simulink model "Sim2Real_ankle_motion_2025a"  (R2025a)
settings: Solver=FixedStepDiscrete  StartTime=0.0  StopTime=8  FixedStep=Ts_1ms  MaxStep=0.002  RelTol=1e-3
InitFcn:
  | modelFile = get_param(bdroot,'FileName');
  | if isempty(modelFile)
  |     error('The model must be saved before running InitFcn.');
  | end
  | 
  | % Folder where the .slx model is located
  | modelFolder = fileparts(char(modelFile));
  | 
  | % Find the parent folder named "resources" by going upwards
  | currentFolder  = modelFolder;
  | materialFolder = '';
  | 
  | while true
  |     [parentFolder, currentName] = fileparts(currentFolder);
  | 
  |     if strcmpi(currentName, 'resources')
  |         materialFolder = currentFolder;
  |         break;
  |     end
  | 
  |     if strcmp(parentFolder, currentFolder)
  |         error('Could not find a parent folder named "resources" starting from: %s', modelFolder);
  |     end
  | 
  |     currentFolder = parentFolder;
  | end
  | 
  | % Search recursively for the MuJoCo XML inside "material"
  | xmlSearch = dir(fullfile(materialFolder, '**', 'unitree_G1.xml'));
  | 
  | if isempty(xmlSearch)
  |     error('MuJoCo XML file not found inside material folder: %s', materialFolder);
  | elseif numel(xmlSearch) > 1
  |     error('Multiple unitree_G1.xml files found inside material folder. Leave only one valid XML.');
  | end
  | 
  | mujocoFolder = xmlSearch(1).folder;
  | xmlFullPath  = fullfile(xmlSearch(1).folder, xmlSearch(1).name);
  | 
  | % Save in base workspace in case you want to inspect them
  | assignin('base','modelFolder',modelFolder);
  | assignin('base','materialFolder',materialFolder);
  | assignin('base','mujocoFolder',mujocoFolder);
  | assignin('base','xmlFullPath',xmlFullPath);
  | 
  | % Final existence check
  | if exist(xmlFullPath,'file') ~= 2
  |     error('MuJoCo XML file not found: %s', xmlFullPath);
  | end
  | 
  | % Add the XML folder to the path so WHICH can find it
  | addpath(mujocoFolder, '-begin');
  | rehash path;
  | 
  | % Run launcher from the same folder as the model
  | launcherFile = fullfile(modelFolder, 'launcher_ankle_motion.mlx');
  | if exist(launcherFile,'file') == 2
  |     run(launcherFile);
  | else
  |     error('Launcher file not found: %s', launcherFile);
  | ... (+17 lines)
StopFcn:
  | drawnow; pause(0.05);
  | 
  | % Stop figures
  | tags = {'G1_IMUState','G1_MotorState'};
  | for k = 1:numel(tags)
  |     delete(findall(0,'Type','uifigure','Tag',tags{k}));
  |     delete(findall(0,'Type','figure' , 'Tag',tags{k}));
  | end
  | 
  | 
  | % Automatic ankle metrics CSV (installed once)
  | addpath(fileparts(get_param('Sim2Real_ankle_motion_2025a', 'FileName')));
  | ankle_motion_csv('save');
undefined symbols (not defined in the file or in its folder): crc, DiscIntNeverNeededParam, mode_machine, mode_pr, motor_cmd, reserve, Ts_1ms
libraries: ros2lib x3, slpidlib x1, mjLib x1
(part 2 of 2)

== matlab function Sim2Real_ankle_motion_2025a/SIM2REAL VARIANT SUBSYSTEM/ROS 2 SUBSYSTEM/ROS 2 SUBSYSTEM/JOINT COMMAND/BUILD motor_cmd BUS ==
  data: motor_cmd output Bus: SL_Bus_unitree_hg_MotorCmd; bus_tau_ref input Bus: bus_tau_ref; bus_pos_ref input Bus: bus_pos_ref; bus_vel_ref input Bus: bus_vel_ref; bus_kp_kd_dyn input Bus: bus_kp_kd_dyn
function motor_cmd = g1_build_motorcmd_vectors( ...
    bus_tau_ref, bus_pos_ref, bus_vel_ref, bus_kp_kd_dyn)
%#codegen

N     = int32(35);   
NBODY = int32(29);   
NLL = int32(6);   % left leg
NRL = int32(6);   % right leg
NW  = int32(3);   % waist
NLA = int32(7);   % left arm
NRA = int32(7);   % right arm

% tau refs
left_leg_tau_ref   = bus_tau_ref.left_leg_tau_ref;
right_leg_tau_ref  = bus_tau_ref.right_leg_tau_ref;
waist_tau_ref      = bus_tau_ref.waist_tau_ref;
left_arm_tau_ref   = bus_tau_ref.left_arm_tau_ref;
right_arm_tau_ref  = bus_tau_ref.right_arm_tau_ref;

% pos refs
left_leg_pos_ref   = bus_pos_ref.left_leg_pos_ref;
right_leg_pos_ref  = bus_pos_ref.right_leg_pos_ref;
waist_pos_ref      = bus_pos_ref.waist_pos_ref;
left_arm_pos_ref   = bus_pos_ref.left_arm_pos_ref;
right_arm_pos_ref  = bus_pos_ref.right_arm_pos_ref;

% vel refs
left_leg_vel_ref   = bus_vel_ref.left_leg_vel_ref;
right_leg_vel_ref  = bus_vel_ref.right_leg_vel_ref;
waist_vel_ref      = bus_vel_ref.waist_vel_ref;
left_arm_vel_ref   = bus_vel_ref.left_arm_vel_ref;
right_arm_vel_ref  = bus_vel_ref.right_arm_vel_ref;

% gains
left_leg_kp_kd     = bus_kp_kd_dyn.left_leg_kp_kd_dyn;
right_leg_kp_kd    = bus_kp_kd_dyn.right_leg_kp_kd_dyn;
waist_kp_kd        = bus_kp_kd_dyn.waist_kp_kd_dyn;
left_arm_kp_kd     = bus_kp_kd_dyn.left_arm_kp_kd_dyn;
right_arm_kp_kd    = bus_kp_kd_dyn.right_arm_kp_kd_dyn;

% Force shapes (column) and types
ll_q   = single(left_leg_pos_ref(:));   rl_q   = single(right_leg_pos_ref(:));
w_q    = single(waist_pos_ref(:));
la_q   = single(left_arm_pos_ref(:));   ra_q   = single(right_arm_pos_ref(:));

ll_dq  = single(left_leg_vel_ref(:));   rl_dq  = single(right_leg_vel_ref(:));
w_dq   = single(waist_vel_ref(:));
la_dq  = single(left_arm_vel_ref(:));   ra_dq  = single(right_arm_vel_ref(:));

ll_tau = single(left_leg_tau_ref(:));   rl_tau = single(right_leg_tau_ref(:));
w_tau  = single(waist_tau_ref(:));
la_tau = single(left_arm_tau_ref(:));   ra_tau = single(right_arm_tau_ref(:));

% Validate input sizes 
ok_ll = (int32(numel(ll_q))  == NLL) && (int32(numel(ll_dq))  == NLL) && (int32(numel(ll_tau))  == NLL);
ok_rl = (int32(numel(rl_q))  == NRL) && (int32(numel(rl_dq))  == NRL) && (int32(numel(rl_tau))  == NRL);
ok_w  = (int32(numel(w_q))   == NW ) && (int32(numel(w_dq))   == NW ) && (int32(numel(w_tau))   == NW );
ok_la = (int32(numel(la_q))  == NLA) && (int32(numel(la_dq))  == NLA) && (int32(numel(la_tau))  == NLA);
ok_ra = (int32(numel(ra_q))  == NRA) && (int32(numel(ra_dq))  == NRA) && (int32(numel(ra_tau))  == NRA);

% Gains: (6x2,6x2,3x2,7x2,7x2) -> 29 
ll_kp = get_col_or_default(left_leg_kp_kd,  1, NLL, single(60));  ll_kd = get_col_or_default(left_leg_kp_kd,  2, NLL, single(1));
rl_kp = get_col_or_default(right_leg_kp_kd, 1, NRL, single(60));  rl_kd = get_col_or_default(right_leg_kp_kd, 2, NRL, single(1));
w_kp  = get_col_or_default(waist_kp_kd,     1, NW,  single(40));  w_kd  = get_col_or_default(waist_kp_kd,     2, NW,  single(1));
la_kp = get_col_or_default(left_arm_kp_kd,  1, NLA, single(40));  la_kd = get_col_or_default(left_arm_kp_kd,  2, NLA, single(1));
ra_kp = get_col_or_default(right_arm_kp_kd, 1, NRA, single(40));  ra_kd = get_col_or_default(right_arm_kp_kd, 2, NRA, single(1));

% Concatenate BODY ONLY (29) 
q_body   = [fix_len(ll_q,NLL);  fix_len(rl_q,NRL);  fix_len(w_q,NW);  fix_len(la_q,NLA);  fix_len(ra_q,NRA)];
dq_body  = [fix_len(ll_dq,NLL); fix_len(rl_dq,NRL); fix_len(w_dq,NW); fix_len(la_dq,NLA); fix_len(ra_dq,NRA)];
tau_body = [fix_len(ll_tau,NLL);fix_len(rl_tau,NRL);fix_len(w_tau,NW); fix_len(la_tau,NLA);fix_len(ra_tau,NRA)];
kp_body  = [fix_len(ll_kp,NLL); fix_len(rl_kp,NRL); fix_len(w_kp,NW);  fix_len(la_kp,NLA); fix_len(ra_kp,NRA)];
kd_body  = [fix_len(ll_kd,NLL); fix_len(rl_kd,NRL); fix_len(w_kd,NW);  fix_len(la_kd,NLA); fix_len(ra_kd,NRA)];

M = int32(numel(q_body));
if M > NBODY
    M = NBODY; %#ok<NASGU>
end

motor_cmd = repmat( ...
    struct( ...
        'mode',    uint8(0), ...
        'q',       single(0), ...
        'dq',      single(0), ...
        'tau',     single(0), ...
        'kp',      single(0), ...
        'kd',      single(0), ...
        'reserve', uint32(0) ...
    ), ...
    double(N), 1);

% Left leg (1..6) 
if ok_ll
    for i = 1:6
        motor_cmd(i).mode    = uint8(1);
        motor_cmd(i).q       = q_body(i);
        motor_cmd(i).dq      = dq_body(i);
        motor_cmd(i).tau     = tau_body(i);
        motor_cmd(i).kp      = kp_body(i);
        motor_cmd(i).kd      = kd_body(i);
        motor_cmd(i).reserve = uint32(0);
    end
end

% Right leg (7..12)
if ok_rl
    for i = 7:12
        motor_cmd(i).mode    = uint8(1);
        motor_cmd(i).q       = q_body(i);
        motor_cmd(i).dq      = dq_body(i);
        motor_cmd(i).tau     = tau_body(i);
        motor_cmd(i).kp      = kp_body(i);
        motor_cmd(i).kd      = kd_body(i);
        motor_cmd(i).reserve = uint32(0);
    end
end

% Waist (13..15) 
if ok_w
    for i = 13:15
        motor_cmd(i).mode    = uint8(1);
        motor_cmd(i).q       = q_body(i);
        motor_cmd(i).dq      = dq_body(i);
        motor_cmd(i).tau     = tau_body(i);
        motor_cmd(i).kp      = kp_body(i);
        motor_cmd(i).kd      = kd_body(i);
        motor_cmd(i).reserve = uint32(0);
    end
end

% Left arm (16..22)
if ok_la
    for i = 16:22
        motor_cmd(i).mode    = uint8(1);
        motor_cmd(i).q       = q_body(i);
        motor_cmd(i).dq      = dq_body(i);
        motor_cmd(i).tau     = tau_body(i);
        motor_cmd(i).kp      = kp_body(i);
        motor_cmd(i).kd      = kd_body(i);
        motor_cmd(i).reserve = uint32(0);
    end
end

% Right arm (23..29)
if ok_ra
    for i = 23:29
        motor_cmd(i).mode    = uint8(1);
        motor_cmd(i).q       = q_body(i);
        motor_cmd(i).dq      = dq_body(i);
        motor_cmd(i).tau     = tau_body(i);
        motor_cmd(i).kp      = kp_body(i);
        motor_cmd(i).kd      = kd_body(i);
        motor_cmd(i).reserve = uint32(0);
    end
end

motor_cmd(14).mode = uint8(0);  % waist roll  (index 13)
motor_cmd(15).mode = uint8(0);  % waist pitch (index 14)

end

function y = fix_len(x, L)
y = zeros(double(L),1,'single');
n = int32(numel(x));
m = n;
if m > L
    m = L;
end
if m > 0
    y(1:double(m)) = x(1:double(m));
end
end

function v = get_col_or_default(M, col, L, default_val)
v = default_val * ones(double(L),1,'single');
if ~isempty(M) && (size(M,2) >= col)
    tmp = single(M(:,col));
    n = int32(numel(tmp));
    m = n;
    if m > L
        m = L;
    end
    if m > 0
        v(1:double(m)) = tmp(1:double(m));
    end
end
end

== matlab function Sim2Real_ankle_motion_2025a/SIM2REAL VARIANT SUBSYSTEM/ROS 2 SUBSYSTEM/ROS 2 SUBSYSTEM/JOINT COMMAND/BUILD CRC ==
  data: cmd_in input; crc_out output
function crc_out = g1_crc_lowcmd_optionA(cmd_in)
%#codegen

N = 35;          
PACK_LEN = 1004; 
cmd = cmd_in;
cmd.crc = uint32(0);
pack = zeros(PACK_LEN, 1, 'uint8');
k = int32(1);

% ---- '<2B2x' ----
pack(k) = uint8(cmd.mode_pr);      k = k + 1;
pack(k) = uint8(cmd.mode_machine); k = k + 1;
pack(k) = uint8(0);                k = k + 1;
pack(k) = uint8(0);                k = k + 1;

% ---- 'B3x5fI' * 35 ----
for i = 1:N
    pack(k) = uint8(cmd.motor_cmd(i).mode); k = k + 1;
    % 3x padding
    pack(k) = uint8(0); k = k + 1;
    pack(k) = uint8(0); k = k + 1;
    pack(k) = uint8(0); k = k + 1;
    [pack,k] = write_f32(pack,k, single(cmd.motor_cmd(i).q));
    [pack,k] = write_f32(pack,k, single(cmd.motor_cmd(i).dq));
    [pack,k] = write_f32(pack,k, single(cmd.motor_cmd(i).tau));
    [pack,k] = write_f32(pack,k, single(cmd.motor_cmd(i).kp));
    [pack,k] = write_f32(pack,k, single(cmd.motor_cmd(i).kd));
    [pack,k] = write_u32(pack,k, uint32(cmd.motor_cmd(i).reserve));
end

% ---- '5I' => reserve[4] + crc placeholder ----
for r = 1:4
    [pack,k] = write_u32(pack,k, uint32(cmd.reserve(r)));
end
[pack,k] = write_u32(pack,k, uint32(0)); % crc placeholder

if k ~= int32(PACK_LEN + 1)
    crc_out = uint32(0);
    return;
end

WORDS = 250; % (1004/4) - 1
words = zeros(WORDS,1,'uint32');

for i = 1:WORDS
    base = (i-1)*4;
    b0 = uint32(pack(base+1));
    b1 = bitshift(uint32(pack(base+2)), 8);
    b2 = bitshift(uint32(pack(base+3)), 16);
    b3 = bitshift(uint32(pack(base+4)), 24);
    words(i) = bitor(bitor(b0,b1), bitor(b2,b3));
end

crc_out = crc32_core_unitree(words);
end

function [buf,k] = write_f32(buf,k,v)
b = typecast(single(v), 'uint8');
buf(k:k+3) = b(:);
k = k + 4;
end

function [buf,k] = write_u32(buf,k,v)
b = typecast(uint32(v), 'uint8');
buf(k:k+3) = b(:);
k = k + 4;
end

function crc = crc32_core_unitree(data)
crc  = uint32(4294967295);     % 0xFFFFFFFF
poly = uint32(79764919);       % 0x04C11DB7
MSB  = uint32(2147483648);     % 1<<31

for i = 1:numel(data)
    current = uint32(data(i));
    bit = MSB;
    for b = 1:32
        if bitand(crc, MSB) ~= 0
            crc = bitxor(bitshift(crc,1), poly);
        else
            crc = bitshift(crc,1);
        end
        if bitand(current, bit) ~= 0
            crc = bitxor(crc, poly);
        end
        bit = bitshift(bit, -1);
    end
end
end

== matlab function Sim2Real_ankle_motion_2025a/HIGH LEVEL CONTROLLER - PI/BUILD BUS POS REF ==
  data: q_pitch_ref input; bus_out output Bus: bus_pos_ref; q_roll_ref input
function bus_out = build_pos_ref_bus(q_pitch_ref, q_roll_ref)
%#codegen

    bus_out.left_leg_pos_ref  = zeros(6,1);
    bus_out.right_leg_pos_ref = zeros(6,1);
    bus_out.waist_pos_ref     = zeros(3,1);
    bus_out.left_arm_pos_ref  = zeros(7,1);
    bus_out.right_arm_pos_ref = zeros(7,1);

    % Pitch: mismo signo en ambos tobillos
    bus_out.left_leg_pos_ref(5)  = q_pitch_ref;
    bus_out.right_leg_pos_ref(5) = q_pitch_ref;

    % Roll: signo opuesto entre tobillo izquierdo y derecho
    bus_out.left_leg_pos_ref(6)  =  q_roll_ref;
    bus_out.right_leg_pos_ref(6) = -q_roll_ref;

end

== matlab function Sim2Real_ankle_motion_2025a/SIM2REAL VARIANT SUBSYSTEM/ROS 2 SUBSYSTEM/ROS 2 SUBSYSTEM/JOINT STATE/BUILD G1 STATE BUS ==
  data: msg input Bus: SL_Bus_unitree_hg_LowState; bus_imu output Bus: bus_imu; bus_tau_state output Bus: bus_tau_state; bus_pos_state output Bus: bus_pos_state; bus_vel_state output Bus: bus_vel_state; mode_machine output uint8; mode_pr output uint8
function [bus_imu, bus_tau_state, bus_pos_state, bus_vel_state, ...
          mode_machine, mode_pr] = ...
    pack_g1_lowstate_buses(msg)
%#codegen

% Default outputs

bus_imu       = init_bus_imu();
bus_tau_state = init_bus_tau_state();
bus_pos_state = init_bus_pos_state();
bus_vel_state = init_bus_vel_state();
mode_machine = uint8(0); %#ok<NASGU>
mode_pr      = uint8(0); %#ok<NASGU>

% IMU packed into bus_imu

bus_imu.quat = double(msg.imu_state.quaternion(:));     % [w x y z]
bus_imu.gyro = double(msg.imu_state.gyroscope(:));      % [gx gy gz]
bus_imu.acc  = double(msg.imu_state.accelerometer(:));  % [ax ay az]

% Modes

mode_machine = uint8(msg.mode_machine);
mode_pr      = uint8(msg.mode_pr);

% Motor indices (0-based Unitree ordering)

% Left leg
L_hip_pitch   = int32(0);
L_hip_roll    = int32(1);
L_hip_yaw     = int32(2);
L_knee        = int32(3);
L_ankle_pitch = int32(4);
L_ankle_roll  = int32(5);

% Right leg
R_hip_pitch   = int32(6);
R_hip_roll    = int32(7);
R_hip_yaw     = int32(8);
R_knee        = int32(9);
R_ankle_pitch = int32(10);
R_ankle_roll  = int32(11);

% Waist
W_yaw   = int32(12);
W_roll  = int32(13);
W_pitch = int32(14);

% Left arm
LA_sh_pitch = int32(15);
LA_sh_roll  = int32(16);
LA_sh_yaw   = int32(17);
LA_elbow    = int32(18);
LA_wr_roll  = int32(19);
LA_wr_pitch = int32(20);
LA_wr_yaw   = int32(21);

% Right arm
RA_sh_pitch = int32(22);
RA_sh_roll  = int32(23);
RA_sh_yaw   = int32(24);
RA_elbow    = int32(25);
RA_wr_roll  = int32(26);
RA_wr_pitch = int32(27);
RA_wr_yaw   = int32(28);

% Positions
% Order:
%   leg  = hip_pitch, hip_roll, hip_yaw, knee, ankle_pitch, ankle_roll
%   arm  = shoulder_pitch, shoulder_roll, shoulder_yaw, elbow, wrist_roll, wrist_pitch, wrist_yaw
%   waist= yaw, roll, pitch

bus_pos_state.left_leg_pos_state(:) = [ ...
    safe_q_double(msg.motor_state, L_hip_pitch); ...
    safe_q_double(msg.motor_state, L_hip_roll); ...
    safe_q_double(msg.motor_state, L_hip_yaw); ...
    safe_q_double(msg.motor_state, L_knee); ...
    safe_q_double(msg.motor_state, L_ankle_pitch); ...
    safe_q_double(msg.motor_state, L_ankle_roll)];

bus_pos_state.right_leg_pos_state(:) = [ ...
    safe_q_double(msg.motor_state, R_hip_pitch); ...
    safe_q_double(msg.motor_state, R_hip_roll); ...
    safe_q_double(msg.motor_state, R_hip_yaw); ...
    safe_q_double(msg.motor_state, R_knee); ...
    safe_q_double(msg.motor_state, R_ankle_pitch); ...
    safe_q_double(msg.motor_state, R_ankle_roll)];

bus_pos_state.waist_pos_state(:) = [ ...
    safe_q_double(msg.motor_state, W_yaw); ...
    safe_q_double(msg.motor_state, W_roll); ...
    safe_q_double(msg.motor_state, W_pitch)];

bus_pos_state.left_arm_pos_state(:) = [ ...
    safe_q_double(msg.motor_state, LA_sh_pitch); ...
    safe_q_double(msg.motor_state, LA_sh_roll); ...
    safe_q_double(msg.motor_state, LA_sh_yaw); ...
    safe_q_double(msg.motor_state, LA_elbow); ...
    safe_q_double(msg.motor_state, LA_wr_roll); ...
    safe_q_double(msg.motor_state, LA_wr_pitch); ...
    safe_q_double(msg.motor_state, LA_wr_yaw)];

bus_pos_state.right_arm_pos_state(:) = [ ...
    safe_q_double(msg.motor_state, RA_sh_pitch); ...
    safe_q_double(msg.motor_state, RA_sh_roll); ...
    safe_q_double(msg.motor_state, RA_sh_yaw); ...
    safe_q_double(msg.motor_state, RA_elbow); ...
    safe_q_double(msg.motor_state, RA_wr_roll); ...
    safe_q_double(msg.motor_state, RA_wr_pitch); ...
    safe_q_double(msg.motor_state, RA_wr_yaw)];

% Velocities

bus_vel_state.left_leg_vel_state(:) = [ ...
    safe_dq_double(msg.motor_state, L_hip_pitch); ...
    safe_dq_double(msg.motor_state, L_hip_roll); ...
    safe_dq_double(msg.motor_state, L_hip_yaw); ...
    safe_dq_double(msg.motor_state, L_knee); ...
    safe_dq_double(msg.motor_state, L_ankle_pitch); ...
    safe_dq_double(msg.motor_state, L_ankle_roll)];

bus_vel_state.right_leg_vel_state(:) = [ ...
    safe_dq_double(msg.motor_state, R_hip_pitch); ...
    safe_dq_double(msg.motor_state, R_hip_roll); ...
    safe_dq_double(msg.motor_state, R_hip_yaw); ...
    safe_dq_double(msg.motor_state, R_knee); ...
    safe_dq_double(msg.motor_state, R_ankle_pitch); ...
    safe_dq_double(msg.motor_state, R_ankle_roll)];

bus_vel_state.waist_vel_state(:) = [ ...
    safe_dq_double(msg.motor_state, W_yaw); ...
    safe_dq_double(msg.motor_state, W_roll); ...
    safe_dq_double(msg.motor_state, W_pitch)];

bus_vel_state.left_arm_vel_state(:) = [ ...
    safe_dq_double(msg.motor_state, LA_sh_pitch); ...
    safe_dq_double(msg.motor_state, LA_sh_roll); ...
    safe_dq_double(msg.motor_state, LA_sh_yaw); ...
    safe_dq_double(msg.motor_state, LA_elbow); ...
    safe_dq_double(msg.motor_state, LA_wr_roll); ...
    safe_dq_double(msg.motor_state, LA_wr_pitch); ...
    safe_dq_double(msg.motor_state, LA_wr_yaw)];

bus_vel_state.right_arm_vel_state(:) = [ ...
    safe_dq_double(msg.motor_state, RA_sh_pitch); ...
    safe_dq_double(msg.motor_state, RA_sh_roll); ...
    safe_dq_double(msg.motor_state, RA_sh_yaw); ...
    safe_dq_double(msg.motor_state, RA_elbow); ...
    safe_dq_double(msg.motor_state, RA_wr_roll); ...
    safe_dq_double(msg.motor_state, RA_wr_pitch); ...
    safe_dq_double(msg.motor_state, RA_wr_yaw)];

% Torques

bus_tau_state.left_leg_tau_state(:) = [ ...
    safe_tau_double(msg.motor_state, L_hip_pitch); ...
    safe_tau_double(msg.motor_state, L_hip_roll); ...
    safe_tau_double(msg.motor_state, L_hip_yaw); ...
    safe_tau_double(msg.motor_state, L_knee); ...
    safe_tau_double(msg.motor_state, L_ankle_pitch); ...
    safe_tau_double(msg.motor_state, L_ankle_roll)];

bus_tau_state.right_leg_tau_state(:) = [ ...
    safe_tau_double(msg.motor_state, R_hip_pitch); ...
    safe_tau_double(msg.motor_state, R_hip_roll); ...
    safe_tau_double(msg.motor_state, R_hip_yaw); ...
    safe_tau_double(msg.motor_state, R_knee); ...
    safe_tau_double(msg.motor_state, R_ankle_pitch); ...
    safe_tau_double(msg.motor_state, R_ankle_roll)];

bus_tau_state.waist_tau_state(:) = [ ...
    safe_tau_double(msg.motor_state, W_yaw); ...
    safe_tau_double(msg.motor_state, W_roll); ...
    safe_tau_double(msg.motor_state, W_pitch)];

bus_tau_state.left_arm_tau_state(:) = [ ...
    safe_tau_double(msg.motor_state, LA_sh_pitch); ...
    safe_tau_double(msg.motor_state, LA_sh_roll); ...
    safe_tau_double(msg.motor_state, LA_sh_yaw); ...
    safe_tau_double(msg.motor_state, LA_elbow); ...
    safe_tau_double(msg.motor_state, LA_wr_roll); ...
    safe_tau_double(msg.motor_state, LA_wr_pitch); ...
    safe_tau_double(msg.motor_state, LA_wr_yaw)];

bus_tau_state.right_arm_tau_state(:) = [ ...
    safe_tau_double(msg.motor_state, RA_sh_pitch); ...
    safe_tau_double(msg.motor_state, RA_sh_roll); ...
    safe_tau_double(msg.motor_state, RA_sh_yaw); ...
    safe_tau_double(msg.motor_state, RA_elbow); ...
    safe_tau_double(msg.motor_state, RA_wr_roll); ...
    safe_tau_double(msg.motor_state, RA_wr_pitch); ...
    safe_tau_double(msg.motor_state, RA_wr_yaw)];

end

function bus_imu = init_bus_imu()
%#codegen
bus_imu.acc  = zeros(3,1);
bus_imu.gyro = zeros(3,1);
bus_imu.quat = zeros(4,1);
end

function bus_tau_state = init_bus_tau_state()
%#codegen
bus_tau_state.left_leg_tau_state   = zeros(6,1);
bus_tau_state.right_leg_tau_state  = zeros(6,1);
bus_tau_state.waist_tau_state      = zeros(3,1);
bus_tau_state.left_arm_tau_state   = zeros(7,1);
bus_tau_state.right_arm_tau_state  = zeros(7,1);
end

function bus_pos_state = init_bus_pos_state()
%#codegen
bus_pos_state.left_leg_pos_state   = zeros(6,1);
bus_pos_state.right_leg_pos_state  = zeros(6,1);
bus_pos_state.waist_pos_state      = zeros(3,1);
bus_pos_state.left_arm_pos_state   = zeros(7,1);
bus_pos_state.right_arm_pos_state  = zeros(7,1);
end

function bus_vel_state = init_bus_vel_state()
%#codegen
bus_vel_state.left_leg_vel_state   = zeros(6,1);
bus_vel_state.right_leg_vel_state  = zeros(6,1);
bus_vel_state.waist_vel_state      = zeros(3,1);
bus_vel_state.left_arm_vel_state   = zeros(7,1);
bus_vel_state.right_arm_vel_state  = zeros(7,1);
end

function v = safe_q_double(motor_state, i0)
N = length(motor_state);
if (i0 >= 0) && (i0 < N)
    v = double(motor_state(i0+1).q);
else
    v = 0.0;
end
end

function v = safe_dq_double(motor_state, i0)
N = length(motor_state);
if (i0 >= 0) && (i0 < N)
    v = double(motor_state(i0+1).dq);
else
    v = 0.0;
end
end

function v = safe_tau_double(motor_state, i0)
N = length(motor_state);
if (i0 >= 0) && (i0 < N)
    v = double(motor_state(i0+1).tau_est);
else
    v = 0.0;
end
end

== matlab function Sim2Real_ankle_motion_2025a/SIM2REAL VARIANT SUBSYSTEM/MuJoCo SUBSYSTEM/MuJoCo SUBSYSTEM/JOINT STATE/BUILD STATE BUSES ==
  data: bus_mujoco_state input Bus: mj_bus_sensor_13323796724550544295; bus_imu output Bus: bus_imu; bus_tau_state output Bus: bus_tau_state; bus_pos_state output Bus: bus_pos_state; bus_vel_state output Bus: bus_vel_state
function [bus_imu, bus_tau_state, bus_pos_state, bus_vel_state] = ...
    mujoco_state_to_internal_buses(bus_mujoco_state)
%#codegen

% Default outputs

bus_imu       = init_bus_imu();
bus_tau_state = init_bus_tau_state();
bus_pos_state = init_bus_pos_state();
bus_vel_state = init_bus_vel_state();

% IMU

bus_imu.quat = double(bus_mujoco_state.imu_quat(:));
bus_imu.gyro = double(bus_mujoco_state.imu_gyro(:));
bus_imu.acc  = double(bus_mujoco_state.imu_acc(:));


% Position-state bus
% Order:
%   leg  = hip_pitch, hip_roll, hip_yaw, knee, ankle_pitch, ankle_roll
%   waist= yaw, roll, pitch
%   arm  = shoulder_pitch, shoulder_roll, shoulder_yaw, elbow, wrist_roll, wrist_pitch, wrist_yaw

bus_pos_state.left_leg_pos_state = [ ...
    double(bus_mujoco_state.left_hip_pitch_pos); ...
    double(bus_mujoco_state.left_hip_roll_pos); ...
    double(bus_mujoco_state.left_hip_yaw_pos); ...
    double(bus_mujoco_state.left_knee_pos); ...
    double(bus_mujoco_state.left_ankle_pitch_pos); ...
    double(bus_mujoco_state.left_ankle_roll_pos)];

bus_pos_state.right_leg_pos_state = [ ...
    double(bus_mujoco_state.right_hip_pitch_pos); ...
    double(bus_mujoco_state.right_hip_roll_pos); ...
    double(bus_mujoco_state.right_hip_yaw_pos); ...
    double(bus_mujoco_state.right_knee_pos); ...
    double(bus_mujoco_state.right_ankle_pitch_pos); ...
    double(bus_mujoco_state.right_ankle_roll_pos)];

bus_pos_state.waist_pos_state = [ ...
    double(bus_mujoco_state.waist_yaw_pos); ...
    double(bus_mujoco_state.waist_roll_pos); ...
    double(bus_mujoco_state.waist_pitch_pos)];

bus_pos_state.left_arm_pos_state = [ ...
    double(bus_mujoco_state.left_shoulder_pitch_pos); ...
    double(bus_mujoco_state.left_shoulder_roll_pos); ...
    double(bus_mujoco_state.left_shoulder_yaw_pos); ...
    double(bus_mujoco_state.left_elbow_pos); ...
    double(bus_mujoco_state.left_wrist_roll_pos); ...
    double(bus_mujoco_state.left_wrist_pitch_pos); ...
    double(bus_mujoco_state.left_wrist_yaw_pos)];

bus_pos_state.right_arm_pos_state = [ ...
    double(bus_mujoco_state.right_shoulder_pitch_pos); ...
    double(bus_mujoco_state.right_shoulder_roll_pos); ...
    double(bus_mujoco_state.right_shoulder_yaw_pos); ...
    double(bus_mujoco_state.right_elbow_pos); ...
    double(bus_mujoco_state.right_wrist_roll_pos); ...
    double(bus_mujoco_state.right_wrist_pitch_pos); ...
    double(bus_mujoco_state.right_wrist_yaw_pos)];

% Velocity-state bus

bus_vel_state.left_leg_vel_state = [ ...
    double(bus_mujoco_state.left_hip_pitch_vel); ...
    double(bus_mujoco_state.left_hip_roll_vel); ...
    double(bus_mujoco_state.left_hip_yaw_vel); ...
    double(bus_mujoco_state.left_knee_vel); ...
    double(bus_mujoco_state.left_ankle_pitch_vel); ...
    double(bus_mujoco_state.left_ankle_roll_vel)];

bus_vel_state.right_leg_vel_state = [ ...
    double(bus_mujoco_state.right_hip_pitch_vel); ...
    double(bus_mujoco_state.right_hip_roll_vel); ...
    double(bus_mujoco_state.right_hip_yaw_vel); ...
    double(bus_mujoco_state.right_knee_vel); ...
    double(bus_mujoco_state.right_ankle_pitch_vel); ...
    double(bus_mujoco_state.right_ankle_roll_vel)];

bus_vel_state.waist_vel_state = [ ...
    double(bus_mujoco_state.waist_yaw_vel); ...
    double(bus_mujoco_state.waist_roll_vel); ...
    double(bus_mujoco_state.waist_pitch_vel)];

bus_vel_state.left_arm_vel_state = [ ...
    double(bus_mujoco_state.left_shoulder_pitch_vel); ...
    double(bus_mujoco_state.left_shoulder_roll_vel); ...
    double(bus_mujoco_state.left_shoulder_yaw_vel); ...
    double(bus_mujoco_state.left_elbow_vel); ...
    double(bus_mujoco_state.left_wrist_roll_vel); ...
    double(bus_mujoco_state.left_wrist_pitch_vel); ...
    double(bus_mujoco_state.left_wrist_yaw_vel)];

bus_vel_state.right_arm_vel_state = [ ...
    double(bus_mujoco_state.right_shoulder_pitch_vel); ...
    double(bus_mujoco_state.right_shoulder_roll_vel); ...
    double(bus_mujoco_state.right_shoulder_yaw_vel); ...
    double(bus_mujoco_state.right_elbow_vel); ...
    double(bus_mujoco_state.right_wrist_roll_vel); ...
    double(bus_mujoco_state.right_wrist_pitch_vel); ...
    double(bus_mujoco_state.right_wrist_yaw_vel)];

% Torque-state bus

bus_tau_state.left_leg_tau_state = [ ...
    double(bus_mujoco_state.left_hip_pitch_torque); ...
    double(bus_mujoco_state.left_hip_roll_torque); ...
    double(bus_mujoco_state.left_hip_yaw_torque); ...
    double(bus_mujoco_state.left_knee_torque); ...
    double(bus_mujoco_state.left_ankle_pitch_torque); ...
    double(bus_mujoco_state.left_ankle_roll_torque)];

bus_tau_state.right_leg_tau_state = [ ...
    double(bus_mujoco_state.right_hip_pitch_torque); ...
    double(bus_mujoco_state.right_hip_roll_torque); ...
    double(bus_mujoco_state.right_hip_yaw_torque); ...
    double(bus_mujoco_state.right_knee_torque); ...
    double(bus_mujoco_state.right_ankle_pitch_torque); ...
    double(bus_mujoco_state.right_ankle_roll_torque)];

bus_tau_state.waist_tau_state = [ ...
    double(bus_mujoco_state.waist_yaw_torque); ...
    double(bus_mujoco_state.waist_roll_torque); ...
    double(bus_mujoco_state.waist_pitch_torque)];

bus_tau_state.left_arm_tau_state = [ ...
    double(bus_mujoco_state.left_shoulder_pitch_torque); ...
    double(bus_mujoco_state.left_shoulder_roll_torque); ...
    double(bus_mujoco_state.left_shoulder_yaw_torque); ...
    double(bus_mujoco_state.left_elbow_torque); ...
    double(bus_mujoco_state.left_wrist_roll_torque); ...
    double(bus_mujoco_state.left_wrist_pitch_torque); ...
    double(bus_mujoco_state.left_wrist_yaw_torque)];

bus_tau_state.right_arm_tau_state = [ ...
    double(bus_mujoco_state.right_shoulder_pitch_torque); ...
    double(bus_mujoco_state.right_shoulder_roll_torque); ...
    double(bus_mujoco_state.right_shoulder_yaw_torque); ...
    double(bus_mujoco_state.right_elbow_torque); ...
    double(bus_mujoco_state.right_wrist_roll_torque); ...
    double(bus_mujoco_state.right_wrist_pitch_torque); ...
    double(bus_mujoco_state.right_wrist_yaw_torque)];

end

% Bus initializers

function bus_imu = init_bus_imu()
%#codegen
bus_imu.acc  = zeros(3,1);
bus_imu.gyro = zeros(3,1);
bus_imu.quat = zeros(4,1);
end

function bus_tau_state = init_bus_tau_state()
%#codegen
bus_tau_state.left_leg_tau_state   = zeros(6,1);
bus_tau_state.right_leg_tau_state  = zeros(6,1);
bus_tau_state.waist_tau_state      = zeros(3,1);
bus_tau_state.left_arm_tau_state   = zeros(7,1);
bus_tau_state.right_arm_tau_state  = zeros(7,1);
end

function bus_pos_state = init_bus_pos_state()
%#codegen
bus_pos_state.left_leg_pos_state   = zeros(6,1);
bus_pos_state.right_leg_pos_state  = zeros(6,1);
bus_pos_state.waist_pos_state      = zeros(3,1);
bus_pos_state.left_arm_pos_state   = zeros(7,1);
bus_pos_state.right_arm_pos_state  = zeros(7,1);
end

function bus_vel_state = init_bus_vel_state()
%#codegen
bus_vel_state.left_leg_vel_state   = zeros(6,1);
bus_vel_state.right_leg_vel_state  = zeros(6,1);
bus_vel_state.waist_vel_state      = zeros(3,1);
bus_vel_state.left_arm_vel_state   = zeros(7,1);
bus_vel_state.right_arm_vel_state  = zeros(7,1);
end

== matlab function Sim2Real_ankle_motion_2025a/SIM2REAL VARIANT SUBSYSTEM/MuJoCo SUBSYSTEM/MuJoCo SUBSYSTEM/JOINT STATE/JOINT TABLE ==
  settings: updateMethod=DISCRETE
  data: bus_tau_state input Bus: bus_tau_state; bus_pos_state input Bus: bus_pos_state; bus_vel_state input; P_MACHINE_DATA parameter
function joints_table_state(bus_tau_state, bus_pos_state, bus_vel_state, P_MACHINE_DATA)
%#codegen

coder.extrinsic('uifigure','uitable','isvalid','set');

persistent F TBL inited jointNames colNames dataCell

if ~(P_MACHINE_DATA.active_states_table ~= 0)
    return;
end

if isempty(inited)
    jointNames = { ...
        'left hip pitch'; ...
        'left hip roll'; ...
        'left hip yaw'; ...
        'left knee'; ...
        'left ankle pitch'; ...
        'left ankle roll'; ...
        'right hip pitch'; ...
        'right hip roll'; ...
        'right hip yaw'; ...
        'right knee'; ...
        'right ankle pitch'; ...
        'right ankle roll'; ...
        'waist yaw'; ...
        'waist roll'; ...
        'waist pitch'; ...
        'left shoulder pitch'; ...
        'left shoulder roll'; ...
        'left shoulder yaw'; ...
        'left elbow'; ...
        'left wrist roll'; ...
        'left wrist pitch'; ...
        'left wrist yaw'; ...
        'right shoulder pitch'; ...
        'right shoulder roll'; ...
        'right shoulder yaw'; ...
        'right elbow'; ...
        'right wrist roll'; ...
        'right wrist pitch'; ...
        'right wrist yaw'; ...
        'left hand thumb 0'; ...
        'left hand thumb 1'; ...
        'left hand thumb 2'; ...
        'left hand middle 0'; ...
        'left hand middle 1'; ...
        'left hand index 0'; ...
        'left hand index 1'; ...
        'right hand thumb 0'; ...
        'right hand thumb 1'; ...
        'right hand thumb 2'; ...
        'right hand middle 0'; ...
        'right hand middle 1'; ...
        'right hand index 0'; ...
        'right hand index 1' ...
    };

    colNames = {'Joint','Torque [N*m]','Velocity [rad/s]','Position [rad]'};
    dataCell = cell(43,4);
    for i = 1:43
        dataCell{i,1} = jointNames{i};
        dataCell{i,2} = 0;
        dataCell{i,3} = 0;
        dataCell{i,4} = 0;
    end

    F = uifigure('Name','Motor State','Position',[120 120 760 760], 'Tag','G1_MotorState');
    TBL = uitable(F, ...
        'Position',[10 10 740 740], ...
        'Data', dataCell, ...
        'RowName', {}, ...
        'ColumnEditable', [false false false false], ...
        'ColumnWidth', {230, 'auto', 'auto', 'auto'}, ...
        'ColumnName', colNames);
    inited = true;
end

% tau
LeftLeg_tau   = clampN(bus_tau_state.left_leg_tau_state,   6);
RightLeg_tau  = clampN(bus_tau_state.right_leg_tau_state,  6);
Waist_tau     = clampN(bus_tau_state.waist_tau_state,      3);
LeftArm_tau   = clampN(bus_tau_state.left_arm_tau_state,   7);
RightArm_tau  = clampN(bus_tau_state.right_arm_tau_state,  7);

% vel
LeftLeg_vel   = clampN(bus_vel_state.left_leg_vel_state,   6);
RightLeg_vel  = clampN(bus_vel_state.right_leg_vel_state,  6);
Waist_vel     = clampN(bus_vel_state.waist_vel_state,      3);
LeftArm_vel   = clampN(bus_vel_state.left_arm_vel_state,   7);
RightArm_vel  = clampN(bus_vel_state.right_arm_vel_state,  7);

% pos
LeftLeg_pos   = clampN(bus_pos_state.left_leg_pos_state,   6);
RightLeg_pos  = clampN(bus_pos_state.right_leg_pos_state,  6);
Waist_pos     = clampN(bus_pos_state.waist_pos_state,      3);
LeftArm_pos   = clampN(bus_pos_state.left_arm_pos_state,   7);
RightArm_pos  = clampN(bus_pos_state.right_arm_pos_state,  7);

% Hands not present in current buses -> zeros
LeftHand_tau  = zeros(7,1);
LeftHand_vel  = zeros(7,1);
LeftHand_pos  = zeros(7,1);
RightHand_tau = zeros(7,1);
RightHand_vel = zeros(7,1);
RightHand_pos = zeros(7,1);

data = [ ...
    LeftLeg_tau,   LeftLeg_vel,   LeftLeg_pos; ...
    RightLeg_tau,  RightLeg_vel,  RightLeg_pos; ...
    Waist_tau,     Waist_vel,     Waist_pos; ...
    LeftArm_tau,   LeftArm_vel,   LeftArm_pos; ...
    RightArm_tau,  RightArm_vel,  RightArm_pos; ...
    LeftHand_tau,  LeftHand_vel,  LeftHand_pos; ...
    RightHand_tau, RightHand_vel, RightHand_pos ];
vals = round3(data);

if ~isempty(F) && ~isempty(TBL) && isvalid(F) && isvalid(TBL)
    for i = 1:43
        dataCell{i,2} = vals(i,1);
        dataCell{i,3} = vals(i,2);
        dataCell{i,4} = vals(i,3);
    end
    set(TBL,'Data', dataCell);
end
end

function v = clampN(x, n)
x = reshape(double(x), [], 1);
m = min(n, numel(x));
v = zeros(n,1);
if m > 0
    v(1:m,1) = x(1:m);
end
end

function y = round3(x)
f = 1000.0;
y = sign(x) .* floor(abs(x).*f + 0.5) ./ f;
end

== matlab function Sim2Real_ankle_motion_2025a/SIM2REAL VARIANT SUBSYSTEM/ROS 2 SUBSYSTEM/ROS 2 SUBSYSTEM/JOINT STATE/IMU GRAPH ==
  settings: updateMethod=DISCRETE
  data: bus_imu input Bus: bus_imu; P_MACHINE_DATA parameter
function imu_graph_function(bus_imu, P_MACHINE_DATA)
%#codegen

coder.extrinsic('figure','subplot','plot3','line','legend','title', ...
                'grid','axis','xlim','ylim','zlim','view','hold','set', ...
                'drawnow','text','xlabel','ylabel');

persistent fig ax3 axA axG ...
           hX hY hZ ...
           la1 la2 la3 ...
           lg1 lg2 lg3 ...
           txtYPR ...
           Tbuf Abuf Gbuf ...
           Nbuf nsamp kbuf ...
           inited ...
           windowSec ...
           Ts_ui ...
           frame_count ...
           orient_div ...
           axis_div ...
           last_xlim_update

if ~(P_MACHINE_DATA.active_IMU_graph ~= 0)
    return;
end

Ts_ui = double(P_MACHINE_DATA.Ts_UIs);
if ~isfinite(Ts_ui) || Ts_ui <= 0
    Ts_ui = 0.05;
end

quat = double(bus_imu.quat(:));   % [w x y z]
gyro = double(bus_imu.gyro(:));   % [rad/s]
acc  = double(bus_imu.acc(:));    % [m/s^2]

if numel(quat) ~= 4 || numel(gyro) ~= 3 || numel(acc) ~= 3
    return;
end

if isempty(inited)
    windowSec = 1.5;
    Nbuf = max(20, ceil(windowSec / Ts_ui) + 3);
    Tbuf = zeros(1, Nbuf);
    Abuf = zeros(3, Nbuf);
    Gbuf = zeros(3, Nbuf);
    nsamp = uint32(0);
    kbuf  = uint32(0);
    frame_count = uint32(0);
    orient_div = uint32(6);   
    axis_div   = uint32(10);  
    last_xlim_update = 0.0;
    fig = figure('Name','IMU State','Position',[80 80 900 900], 'Tag','G1_IMUState');
    ax3 = subplot(3,1,1,'Parent',fig);
    title(ax3, {'IMU frame [quat]'; ' '});
    grid(ax3,'on');
    axis(ax3,'equal');
    xlim(ax3,[-1.1 1.1]);
    ylim(ax3,[-1.1 1.1]);
    zlim(ax3,[-1.1 1.1]);
    view(ax3,55,25);
    hold(ax3,'on');
    plot3(ax3,[-1.1 1.1],[0 0],[0 0],'k:');
    plot3(ax3,[0 0],[-1.1 1.1],[0 0],'k:');
    plot3(ax3,[0 0],[0 0],[-1.1 1.1],'k:');
    hX = plot3(ax3,[0 1],[0 0],[0 0],'LineWidth',3,'Color',[1 0 0]);
    hY = plot3(ax3,[0 0],[0 1],[0 0],'LineWidth',3,'Color',[0 0.5 0]);
    hZ = plot3(ax3,[0 0],[0 0],[0 1],'LineWidth',3,'Color',[0 0 1]);
    text(ax3, 1.675, 0.75, ' IMU frame [RPY]', ...
        'Units','normalized', ...
        'HorizontalAlignment','left', ...
        'FontWeight','bold', ...
        'FontSize',10, ...
        'Clipping','off');
    txtYPR = text(ax3, 1.675, 0.50, ...
        sprintf(['\\color[rgb]{1,0,0}Roll:  %+.2f°\\color{black}\n' ...
         '\\color[rgb]{0,0.5,0}Pitch: %+.2f°\\color{black}\n' ...
         '\\color[rgb]{0,0,1}Yaw:   %+.2f°\\color{black}'],0,0,0), ...
        'Units','normalized', ...
        'HorizontalAlignment','left', ...
        'Interpreter','tex', ...
        'FontWeight','bold', ...
        'BackgroundColor','none', ...
        'Color','k', ...
        'FontName','FixedWidth', ...
        'FontSize',11, ...
        'Clipping','off');
    hold(ax3,'off');
    set(ax3,'Position',[0.05 0.68 0.60 0.25]);

    axA = subplot(3,1,2,'Parent',fig);
    grid(axA,'on');
    title(axA,'Accelerometer');
    ylabel(axA,'Amplitude [m/s^2]');
    xlabel(axA,'Time [s]');
    xlim(axA,[-windowSec 0.0]);
    la1 = line(axA,0,0,'Color',[1 0 0]);
    la2 = line(axA,0,0,'Color',[0 0.5 0]);
    la3 = line(axA,0,0,'Color',[0 0 1]);
    legend(axA,{'ax','ay','az'},'Location','northeastoutside');

    axG = subplot(3,1,3,'Parent',fig);
    grid(axG,'on');
    title(axG,'Gyro');
    xlabel(axG,'Time [s]');
    ylabel(axG,'Amplitude [rad/s]');
    xlim(axG,[-windowSec 0.0]);
    lg1 = line(axG,0,0,'Color',[1 0 0]);
    lg2 = line(axG,0,0,'Color',[0 0.5 0]);
    lg3 = line(axG,0,0,'Color',[0 0 1]);
    legend(axG,{'gx','gy','gz'},'Location','northeastoutside');
    inited = true;
end

kbuf = kbuf + uint32(1);
if kbuf > uint32(Nbuf)
    kbuf = uint32(1);
end
k = double(kbuf);
if nsamp < uint32(Nbuf)
    nsamp = nsamp + uint32(1);
end
n = double(nsamp);
frame_count = frame_count + uint32(1);
if n == 1
    Tbuf(1,k) = 0.0;
else
    if k == 1
        kprev = Nbuf;
    else
        kprev = k - 1;
    end
    Tbuf(1,k) = Tbuf(1,kprev) + Ts_ui;
end
Abuf(:,k) = -acc(:);
Gbuf(:,k) = gyro(:);

if n < Nbuf
    tt = Tbuf(1,1:n);
    aa = Abuf(:,1:n);
    gg = Gbuf(:,1:n);
else
    if k < Nbuf
        ord = [k+1:Nbuf, 1:k];
    else
        ord = 1:Nbuf;
    end
    tt = Tbuf(ord);
    aa = Abuf(:,ord);
    gg = Gbuf(:,ord);
end

if ~isempty(tt)
    tt = tt - tt(end);
end

if mod(double(frame_count), double(orient_div)) == 0
    R  = quat2rotm_wxyz(quat(:)');
    ex = R(:,1);
    ey = R(:,2);
    ez = R(:,3);
    set(hX,'XData',[0 ex(1)],'YData',[0 ex(2)],'ZData',[0 ex(3)]);
    set(hY,'XData',[0 ey(1)],'YData',[0 ey(2)],'ZData',[0 ey(3)]);
    set(hZ,'XData',[0 ez(1)],'YData',[0 ez(2)],'ZData',[0 ez(3)]);
    [yaw,pitch,roll] = quat_to_ypr_zyx(quat(:)');
    set(txtYPR,'String',sprintf([ ...
        '\\color[rgb]{1,0,0}Roll:  %+.2f°\\color{black}\n' ...
        '\\color[rgb]{0,0.5,0}Pitch: %+.2f°\\color{black}\n' ...
        '\\color[rgb]{0,0,1}Yaw:   %+.2f°\\color{black}'], ...
        roll*180/pi, pitch*180/pi, yaw*180/pi));
end

set(la1,'XData',tt,'YData',aa(1,:));
set(la2,'XData',tt,'YData',aa(2,:));
set(la3,'XData',tt,'YData',aa(3,:));
set(lg1,'XData',tt,'YData',gg(1,:));
set(lg2,'XData',tt,'YData',gg(2,:));
set(lg3,'XData',tt,'YData',gg(3,:));

if mod(double(frame_count), double(axis_div)) == 0
    if abs(last_xlim_update - tt(end)) > 0.25 || frame_count == uint32(1)
        xlim(axA,[-windowSec 0.0]);
        xlim(axG,[-windowSec 0.0]);
        last_xlim_update = tt(end);
    end
    ylim_soft_fast(axA, aa);
    ylim_soft_fast(axG, gg);
end
drawnow limitrate nocallbacks;
end

function R = quat2rotm_wxyz(q)
w=q(1); x=q(2); y=q(3); z=q(4);
xx=x*x; yy=y*y; zz=z*z; wx=w*x; wy=w*y; wz=w*z; xy=x*y; xz=x*z; yz=y*z;
R=[1-2*(yy+zz)  2*(xy-wz)  2*(xz+wy);
   2*(xy+wz)  1-2*(xx+zz)  2*(yz-wx);
   2*(xz-wy)  2*(yz+wx)    1-2*(xx+yy)];
end

function [yaw,pitch,roll] = quat_to_ypr_zyx(q)
w=q(1); x=q(2); y=q(3); z=q(4);
yaw   = atan2(2*(w*z + x*y), 1 - 2*(y*y + z*z));
pitch = asin(max(-1,min(1, 2*(w*y - z*x))));
roll  = atan2(2*(w*x + y*z), 1 - 2*(x*x + y*y));
end

function ylim_soft_fast(ax, Y)
if isempty(Y)
    ylim(ax,[-1 1]);
    return;
end

m1 = max(abs(Y(1,:)));
m2 = max(abs(Y(2,:)));
m3 = max(abs(Y(3,:)));
v = max(1e-6, max([m1 m2 m3]));
ylim(ax,[-1.2*v, 1.2*v]);
end

== matlab function Sim2Real_ankle_motion_2025a/SIM2REAL VARIANT SUBSYSTEM/ROS 2 SUBSYSTEM/ROS 2 SUBSYSTEM/JOINT STATE/JOINT TABLE ==
  settings: updateMethod=DISCRETE
  data: bus_tau_state input Bus: bus_tau_state; bus_pos_state input Bus: bus_pos_state; bus_vel_state input; P_MACHINE_DATA parameter
function joints_table_state(bus_tau_state, bus_pos_state, bus_vel_state, P_MACHINE_DATA)
%#codegen

coder.extrinsic('uifigure','uitable','isvalid','set');

persistent F TBL inited jointNames colNames dataCell

if ~(P_MACHINE_DATA.active_states_table ~= 0)
    return;
end

if isempty(inited)
    jointNames = { ...
        'left hip pitch'; ...
        'left hip roll'; ...
        'left hip yaw'; ...
        'left knee'; ...
        'left ankle pitch'; ...
        'left ankle roll'; ...
        'right hip pitch'; ...
        'right hip roll'; ...
        'right hip yaw'; ...
        'right knee'; ...
        'right ankle pitch'; ...
        'right ankle roll'; ...
        'waist yaw'; ...
        'waist roll'; ...
        'waist pitch'; ...
        'left shoulder pitch'; ...
        'left shoulder roll'; ...
        'left shoulder yaw'; ...
        'left elbow'; ...
        'left wrist roll'; ...
        'left wrist pitch'; ...
        'left wrist yaw'; ...
        'right shoulder pitch'; ...
        'right shoulder roll'; ...
        'right shoulder yaw'; ...
        'right elbow'; ...
        'right wrist roll'; ...
        'right wrist pitch'; ...
        'right wrist yaw'; ...
        'left hand thumb 0'; ...
        'left hand thumb 1'; ...
        'left hand thumb 2'; ...
        'left hand middle 0'; ...
        'left hand middle 1'; ...
        'left hand index 0'; ...
        'left hand index 1'; ...
        'right hand thumb 0'; ...
        'right hand thumb 1'; ...
        'right hand thumb 2'; ...
        'right hand middle 0'; ...
        'right hand middle 1'; ...
        'right hand index 0'; ...
        'right hand index 1' ...
    };

    colNames = {'Joint','Torque [N*m]','Velocity [rad/s]','Position [rad]'};
    dataCell = cell(43,4);
    for i = 1:43
        dataCell{i,1} = jointNames{i};
        dataCell{i,2} = 0;
        dataCell{i,3} = 0;
        dataCell{i,4} = 0;
    end

    F = uifigure('Name','Motor State','Position',[120 120 760 760], 'Tag','G1_MotorState');
    TBL = uitable(F, ...
        'Position',[10 10 740 740], ...
        'Data', dataCell, ...
        'RowName', {}, ...
        'ColumnEditable', [false false false false], ...
        'ColumnWidth', {230, 'auto', 'auto', 'auto'}, ...
        'ColumnName', colNames);
    inited = true;
end

% tau
LeftLeg_tau   = clampN(bus_tau_state.left_leg_tau_state,   6);
RightLeg_tau  = clampN(bus_tau_state.right_leg_tau_state,  6);
Waist_tau     = clampN(bus_tau_state.waist_tau_state,      3);
LeftArm_tau   = clampN(bus_tau_state.left_arm_tau_state,   7);
RightArm_tau  = clampN(bus_tau_state.right_arm_tau_state,  7);

% vel
LeftLeg_vel   = clampN(bus_vel_state.left_leg_vel_state,   6);
RightLeg_vel  = clampN(bus_vel_state.right_leg_vel_state,  6);
Waist_vel     = clampN(bus_vel_state.waist_vel_state,      3);
LeftArm_vel   = clampN(bus_vel_state.left_arm_vel_state,   7);
RightArm_vel  = clampN(bus_vel_state.right_arm_vel_state,  7);

% pos
LeftLeg_pos   = clampN(bus_pos_state.left_leg_pos_state,   6);
RightLeg_pos  = clampN(bus_pos_state.right_leg_pos_state,  6);
Waist_pos     = clampN(bus_pos_state.waist_pos_state,      3);
LeftArm_pos   = clampN(bus_pos_state.left_arm_pos_state,   7);
RightArm_pos  = clampN(bus_pos_state.right_arm_pos_state,  7);

% Hands not present in current buses -> zeros
LeftHand_tau  = zeros(7,1);
LeftHand_vel  = zeros(7,1);
LeftHand_pos  = zeros(7,1);
RightHand_tau = zeros(7,1);
RightHand_vel = zeros(7,1);
RightHand_pos = zeros(7,1);

data = [ ...
    LeftLeg_tau,   LeftLeg_vel,   LeftLeg_pos; ...
    RightLeg_tau,  RightLeg_vel,  RightLeg_pos; ...
    Waist_tau,     Waist_vel,     Waist_pos; ...
    LeftArm_tau,   LeftArm_vel,   LeftArm_pos; ...
    RightArm_tau,  RightArm_vel,  RightArm_pos; ...
    LeftHand_tau,  LeftHand_vel,  LeftHand_pos; ...
    RightHand_tau, RightHand_vel, RightHand_pos ];
vals = round3(data);

if ~isempty(F) && ~isempty(TBL) && isvalid(F) && isvalid(TBL)
    for i = 1:43
        dataCell{i,2} = vals(i,1);
        dataCell{i,3} = vals(i,2);
        dataCell{i,4} = vals(i,3);
    end
    set(TBL,'Data', dataCell);
end
end

function v = clampN(x, n)
x = reshape(double(x), [], 1);
m = min(n, numel(x));
v = zeros(n,1);
if m > 0
    v(1:m,1) = x(1:m);
end
end

function y = round3(x)
f = 1000.0;
y = sign(x) .* floor(abs(x).*f + 0.5) ./ f;
end

== matlab function Sim2Real_ankle_motion_2025a/SIM2REAL VARIANT SUBSYSTEM/MuJoCo SUBSYSTEM/MuJoCo SUBSYSTEM/JOINT COMMAND/CRANE ==
  data: start_enable input; crane_tau output; ankle_pitch_tau output; grip_open output; P_MACHINE_DATA parameter
function [crane_tau, ankle_pitch_tau, grip_open] = crane_function(start_enable, P_MACHINE_DATA)

Ts      = P_MACHINE_DATA.Ts_1ms;  
u_hold  = 1250;
u_low   = 440;
u_high  = 730; 
t_wait  = 1.7;
t_kick  = 0.9;
t_ramp  = 2.5;
t_raise = 1.7;
t_pre   = 0.5;
grip_base     = -0.08;      % max value -0.15
grip_hold     =  1.2;       % max value 2.45
grip_wait_SE1 = 10.0;
crane_boost_tau   = 1000;   % 800 to go up, 720 to hold
crane_boost_delay = 0.05;  
crane_boost_time  = 2.0;   

persistent t_elapsed grip_latched se1_steps boost_stage boost_steps

if isempty(t_elapsed)
    t_elapsed    = 0;
    grip_latched = false;
    se1_steps    = uint32(0);
    boost_stage  = uint8(0);
    boost_steps  = uint32(0);
end

if start_enable == 0
    crane_tau       = u_hold;
    ankle_pitch_tau = 0.15;
    grip_open       = grip_base;
    t_elapsed    = 0;
    grip_latched = false;
    se1_steps    = uint32(0);
    boost_stage  = uint8(0);
    boost_steps  = uint32(0);
    return;
end

t1 = t_wait;
t2 = t_wait + t_kick;

if t_elapsed < t1
    ankle_pitch_tau = 0;
elseif t_elapsed < t2
    ankle_pitch_tau = -0.35;
else
    ankle_pitch_tau = 0;
end

if t_elapsed < t_ramp
    alphaA = t_elapsed / t_ramp;   
    if alphaA < 0, alphaA = 0; end
    if alphaA > 1, alphaA = 1; end
    crane_tau = u_hold + (u_low - u_hold) * alphaA;
else
    crane_tau = u_low;
end

t_raise_start = t2 - t_pre;

if t_elapsed >= t_raise_start
    tauB = t_elapsed - t_raise_start;
    if tauB < t_raise
        alphaB = tauB / t_raise;
        if alphaB < 0, alphaB = 0; end
        if alphaB > 1, alphaB = 1; end
        crane_tau = u_low + (u_high - u_low) * alphaB;
    else
        crane_tau = u_high;
    end
end

se1_steps = se1_steps + uint32(1);

if ~grip_latched
    if double(se1_steps) * Ts >= grip_wait_SE1
        grip_latched = true;
        boost_stage = uint8(1); 
        boost_steps = uint32(0);
    end
end

if grip_latched
    grip_open = grip_hold;  
else
    grip_open = grip_base; 
end

if boost_stage ~= uint8(0)
    boost_steps = boost_steps + uint32(1);
    t_boost = double(boost_steps) * Ts;
    if boost_stage == uint8(1)
        % delay stage
        if t_boost >= crane_boost_delay
            boost_stage = uint8(2);
            boost_steps = uint32(0); 
        end
    elseif boost_stage == uint8(2)
        if (double(boost_steps) * Ts) <= crane_boost_time
            crane_tau = crane_boost_tau;
        else
            boost_stage = uint8(0);    
        end
    end
end

t_elapsed = t_elapsed + Ts;
end
